simulink model "aerodynamic_model_V1_2_Wrench"  (R2025b)
settings: Solver=ode4  StartTime=0.0  StopTime=0.3  FixedStep=Ts  RelTol=1e-3
InitFcn:
  | % Run initial_main.m first to load Ad,As,Tq_prop,Tq_mass,...
values from neighbouring files (symbols this model uses):
  alpha_du0_v_tail_L = trim_aero_ic.v_tail_L.alpha_du0    [initial_main_V1_1.m]
  alpha_du0_v_tail_R = trim_aero_ic.v_tail_R.alpha_du0    [initial_main_V1_1.m]
  alpha_du0_wing_L = trim_aero_ic.wing_L.alpha_du0    [initial_main_V1_1.m]
  alpha_du0_wing_R = trim_aero_ic.wing_R.alpha_du0    [initial_main_V1_1.m]
  As = sys_sd.A    [initial_main_V1_1.m]
  BladePitch_deg = 34    [initial_main_V1_1.m]
  Bs = sys_sd.B    [initial_main_V1_1.m]
  Cs = sys_sd.C    [initial_main_V1_1.m]
  ctrl_delta_lim_deg = strips.delta_lim_deg    [initial_main_V1_1.m]
  ctrl_map_aileron_L = aero.wing_L.map_aileron(:)    [initial_main_V1_1.m]
  ctrl_map_aileron_R = aero.wing_R.map_aileron(:)    [initial_main_V1_1.m]
  ctrl_map_tail_L = aero.v_tail_L.map_tail(:)    [initial_main_V1_1.m]
  ctrl_map_tail_R = aero.v_tail_R.map_tail(:)    [initial_main_V1_1.m]
  Ds = sys_sd.D    [initial_main_V1_1.m]
  I_cg_b = R_sb * I_cg_m * R_sb.'    [aeroelastic.m]    (also in initial_main_V1_1.m = grav.I_cg_b)
  I_cg_b_inv = R_sb * I_cg_m_inv * R_sb.'    [aeroelastic.m]    (also in initial_main_V1_1.m = grav.I_cg_b_inv)
  m_node = zeros(n_id, 1)    [aeroelastic.m]    (also in generate_pullup_load_cloud.m = evalin('base', 'm_node(:)'); initial_main_V1_1.m = nodal.m_node)
  m_total_kg = evalin('base', 'm_total_kg')    [generate_pullup_load_cloud.m]    (also in initial_main_V1_1.m = grav.m_total_kg)
  n_modes = size(Phi, 2)    [aeroelastic.m]    (also in initial_main_V1_1.m = n_rigid + n_elastic)
  ones_1_tail = ones(1, size(r_cg2ac_b_v_tail_L, 2))    [initial_main_V1_1.m]
  ones_1_wing = ones(1, size(r_cg2ac_b_wing_L, 2))    [initial_main_V1_1.m]
  Phi = evalin('base', 'Phi')    [generate_pullup_load_cloud.m]    (also in initial_main_V1_1.m = strips.Phi)
  polar_alpha_deg = polar.alpha_deg(:).'    [initial_main_V1_1.m]
  polar_CD = polar.CD(:).'    [initial_main_V1_1.m]
  polar_CDp = polar.CDp(:).'    [initial_main_V1_1.m]
  polar_CL = polar.CL(:).'    [initial_main_V1_1.m]
  polar_CM = polar.CM(:).'    [initial_main_V1_1.m]
  r_cg2ac_b_v_tail_L = R_sb * aero.v_tail_L.r_ac_s    [initial_main_V1_1.m]
  r_cg2ac_b_v_tail_R = R_sb * aero.v_tail_R.r_ac_s    [initial_main_V1_1.m]
  r_cg2ac_b_wing_L = R_sb * aero.wing_L.r_ac_s    [initial_main_V1_1.m]
  r_cg2ac_b_wing_R = R_sb * aero.wing_R.r_ac_s    [initial_main_V1_1.m]
  r_cg2kink_b = eng.r_cg2kink_b    [initial_main_V1_1.m]
  r_cg2node_b = aeroelastic.node_arms(nodes, 'R_sb', R_sb).r_cg2node_b    [initial_main_V1_1.m]
  surface_nodes = aeroelastic.surface_load_nodes(nodes)    [initial_main_V1_1.m]
  T_aero2W = aeroelastic.wing_aileron_to_W(strips).T    [initial_main_V1_1.m]
  T_prop2W = load_maps.T_prop2W    [initial_main_V1_1.m]
  Tq_mass = load_maps.Tq_mass    [initial_main_V1_1.m]
  trim_Attitude_rad0 = trim_default.Attitude_rad0    [initial_main_V1_1.m]
  trim_Omega_b0 = trim_default.Omega_b0    [initial_main_V1_1.m]
  trim_Position0 = trim_default.Position0    [initial_main_V1_1.m]
  trim_Velocity_b0 = trim_default.Velocity_b0    [initial_main_V1_1.m]
  Ts = 0.001    [initial_main_V1_1.m]
  U = 55    [initial_main_V1_1.m]
  v_tail_cant_rad = deg2rad(v_tail_cant_deg)    [initial_main_V1_1.m]
  W_mass_g = grav.W_mass    [initial_main_V1_1.m]
  x0_structure = trim_default.x0_structure    [initial_main_V1_1.m]
  x0_wagner_v_tail_L = trim_aero_ic.v_tail_L.x0_wagner    [initial_main_V1_1.m]
  x0_wagner_v_tail_R = trim_aero_ic.v_tail_R.x0_wagner    [initial_main_V1_1.m]
  x0_wagner_wing_L = trim_aero_ic.wing_L.x0_wagner    [initial_main_V1_1.m]
  x0_wagner_wing_R = trim_aero_ic.wing_R.x0_wagner    [initial_main_V1_1.m]
undefined symbols (not defined in the file or in its folder): Ad_v_tail_L, Ad_v_tail_R, Ad_wing_L, Ad_wing_R, Bd_v_tail_L, Bd_v_tail_R, Bd_wing_L, Bd_wing_R, c_over_2U_v_tail_L, c_over_2U_v_tail_R, c_over_2U_wing_L, c_over_2U_wing_R, Cd_v_tail_L, Cd_v_tail_R, Cd_wing_L, Cd_wing_R, Dd_v_tail_L, Dd_v_tail_R, Dd_wing_L, Dd_wing_R, G_du_v_tail_L, G_du_v_tail_R, G_du_wing_L, G_du_wing_R, polar_aileron_alpha_deg, polar_aileron_dCD, polar_aileron_dCL, polar_aileron_dCM, polar_aileron_delta_deg, polar_ruddervator_alpha_deg, polar_ruddervator_dCD, polar_ruddervator_dCL, polar_ruddervator_dCM, polar_ruddervator_delta_deg, qS_strip_v_tail_L, qS_strip_v_tail_R, qS_strip_wing_L, qS_strip_wing_R, qSc_strip_v_tail_L, qSc_strip_v_tail_R, qSc_strip_wing_L, qSc_strip_wing_R, T_m2b_v_tail_L, T_m2b_v_tail_R, T_m2b_wing_L, T_m2b_wing_R, T_m2h_v_tail_L, T_m2h_v_tail_R, T_m2h_wing_L, T_m2h_wing_R, Tq_CM_v_tail_L, Tq_CM_v_tail_R, Tq_CM_wing_L, Tq_CM_wing_R, Tq_D_v_tail_L, Tq_D_v_tail_R, Tq_D_wing_L, Tq_D_wing_R, Tq_v_tail_L, Tq_v_tail_R ... (+2)
libraries: Prop_gryo x12, matrix_library x2
(part 4 of 6)

== system aerodynamic_model_V1_2_Wrench/Load Estimator/Engine_station/Subsystem7 ==
  In1 : Inport
  r_cg_up : Inport  Port=2
  Bus Creator : BusCreator  Inputs=6
  Bus Creator1 : BusCreator  Inputs=6
  Bus Creator2 : BusCreator  Inputs=6
  Bus Creator4 : BusCreator  Inputs=3
  Constant : Constant  Value=r_cg2node_b(:,67)
  Constant1 : Constant  Value=r_cg2node_b(:,66)
  Constant2 : Constant  Value=0
  Constant3 : Constant  Value=r_cg2node_b(:,46)
  Constant4 : Constant  Value=[0 0 0]/180*pi
  Constant5 : Constant  Value=[-7 0 0]/180*pi
  Constant6 : Constant  Value=-7
  Constant7 : Constant  Value=90
  Demux{1..6} (6 alike) : Demux  Outputs=3
  Gain : Gain  Gain=pi/180
  MATLAB Function1 : MATLAB Function  TreatAsAtomicUnit=on
  MATLAB Function2 : MATLAB Function  TreatAsAtomicUnit=on
  MATLAB Function3 : MATLAB Function  TreatAsAtomicUnit=on
  Mux : Mux  Inputs=3
  Product{1..4,6..7} (6 alike) : Product  Multiplication=Matrix(*)
  Rotation Angles to Direction Cosine Matrix : Angle2Dcm  rotationOrder=XYZ
      settings: AttributesFormatString=Rotation Order: %<rotationOrder>
  Rotation Angles to Direction Cosine Matrix1 : Angle2Dcm  rotationOrder=XYZ
      settings: AttributesFormatString=Rotation Order: %<rotationOrder>
  Rotation Angles to Direction Cosine Matrix2 : Angle2Dcm  rotationOrder=XYZ
      settings: AttributesFormatString=Rotation Order: %<rotationOrder>
  Selector1 : Selector  NumberOfDimensions=2  InputPortWidth=3  IndexOptions=Select all,Index vector (dialog)  Indices=[1:6],[67]  OutputSizes=1,1
  Selector10 : Selector  NumberOfDimensions=2  InputPortWidth=3  IndexOptions=Index vector (dialog),Select all  Indices=[4:6],[surface_nodes.wing_R.node_id]  OutputSizes=1,1
  Selector11 : Selector  NumberOfDimensions=2  InputPortWidth=3  IndexOptions=Index vector (dialog),Select all  Indices=[4:6],[surface_nodes.wing_R.node_id]  OutputSizes=1,1
  Selector12 : Selector  NumberOfDimensions=2  InputPortWidth=3  IndexOptions=Index vector (dialog),Select all  Indices=[1:3],[surface_nodes.wing_R.node_id]  OutputSizes=1,1
  Selector13 : Selector  NumberOfDimensions=2  InputPortWidth=3  IndexOptions=Index vector (dialog),Select all  Indices=[4:6],[surface_nodes.wing_R.node_id]  OutputSizes=1,1
  Selector14 : Selector  NumberOfDimensions=2  InputPortWidth=3  IndexOptions=Index vector (dialog),Select all  Indices=[1:3],[surface_nodes.wing_R.node_id]  OutputSizes=1,1
  Selector2 : Selector  NumberOfDimensions=2  InputPortWidth=3  IndexOptions=Select all,Index vector (dialog)  Indices=[1:6],[66 67]  OutputSizes=1,1
  Selector3 : Selector  NumberOfDimensions=2  InputPortWidth=3  IndexOptions=Select all,Index vector (dialog)  Indices=[1:6],[67]  OutputSizes=1,1
  Selector4 : Selector  NumberOfDimensions=2  InputPortWidth=3  IndexOptions=Select all,Index vector (dialog)  Indices=[1:6],[66 67]  OutputSizes=1,1
  Selector5 : Selector  NumberOfDimensions=2  InputPortWidth=3  IndexOptions=Select all,Index vector (dialog)  Indices=[1:6],[65:67]  OutputSizes=1,1
  Selector6 : Selector  NumberOfDimensions=2  InputPortWidth=3  IndexOptions=Select all,Index vector (dialog)  Indices=[1:6],[65:67]  OutputSizes=1,1
  Selector9 : Selector  NumberOfDimensions=2  InputPortWidth=3  IndexOptions=Index vector (dialog),Select all  Indices=[1:3],[surface_nodes.wing_R.node_id]  OutputSizes=1,1
  Out1 : Outport
  wires:
  Demux3/3 -> Bus Creator2/3  "shear_forcez"
  Selector4/1 -> MATLAB Function2/3(r)
  MATLAB Function3/2(M_b) -> Product4/2
  MATLAB Function1/2(M_b) -> Product7/2
  Demux1/2 -> Bus Creator1/2  "shear_forcey"
  Demux6/3 -> Bus Creator2/6  "Bending_momenty"
  MATLAB Function1/1(F_b) -> Product6/2
  Selector6/1 -> MATLAB Function3/3(r)
  Demux1/3 -> Bus Creator1/3  "shear_forcez"
  Demux5/2 -> Bus Creator/5  "Bending_momentx"
  Selector2/1 -> Selector11/1, Selector12/1
  Demux4/2 -> Bus Creator/2  "shear_forcey"
  Selector12/1 -> MATLAB Function2/1(F)
  Bus Creator1/1 -> Bus Creator4/2
  Demux5/3 -> Bus Creator/6  "Bending_momenty"
  Selector5/1 -> Selector13/1, Selector14/1
  Constant1/1 -> MATLAB Function2/4(p)
  Demux5/1 -> Bus Creator/4  "Torision_moment"
  Constant2/1 -> Mux/3
  Gain/1 -> Rotation Angles to Direction Cosine Matrix/1
  Bus Creator2/1 -> Bus Creator4/3
  Product3/1 -> Demux3/1
  Demux1/1 -> Bus Creator1/1  "Axial_Force"
  Selector9/1 -> MATLAB Function1/1(F)
  Product7/1 -> Demux5/1
  Bus Creator/1 -> Bus Creator4/1
  Demux4/1 -> Bus Creator/1  "Axial_Force"
  In1/1 -> Selector1/1, Selector5/1, Selector2/1
  Demux2/1 -> Bus Creator1/4  "Torision_moment"
  Rotation Angles to Direction Cosine Matrix2/1 -> Product4/1, Product3/1
  Constant6/1 -> Mux/1
  Mux/1 -> Gain/1
  Product6/1 -> Demux4/1
  Demux3/1 -> Bus Creator2/1  "Axial_Force"
  Selector11/1 -> MATLAB Function2/2(M)
  Demux6/1 -> Bus Creator2/4  "Torision_moment"
  Demux2/3 -> Bus Creator1/6  "Bending_momenty"
  MATLAB Function2/1(F_b) -> Product1/2
  Rotation Angles to Direction Cosine Matrix1/1 -> Product1/1, Product2/1
  Demux4/3 -> Bus Creator/3  "shear_forcez"
  Constant3/1 -> MATLAB Function3/4(p)
  Product1/1 -> Demux1/1
  Product2/1 -> Demux2/1
  Constant5/1 -> Rotation Angles to Direction Cosine Matrix1/1
  MATLAB Function2/2(M_b) -> Product2/2
  Bus Creator4/1 -> Out1/1
  r_cg_up/1 -> Selector6/1, Selector4/1, Selector3/1
  Selector1/1 -> Selector10/1, Selector9/1
  MATLAB Function3/1(F_b) -> Product3/2
  Constant7/1 -> Mux/2
  Selector10/1 -> MATLAB Function1/2(M)
  Rotation Angles to Direction Cosine Matrix/1 -> Product7/1, Product6/1
  Selector13/1 -> MATLAB Function3/2(M)
  Constant4/1 -> Rotation Angles to Direction Cosine Matrix2/1
  Selector14/1 -> MATLAB Function3/1(F)
  Demux2/2 -> Bus Creator1/5  "Bending_momentx"
  Demux3/2 -> Bus Creator2/2  "shear_forcey"
  Selector3/1 -> MATLAB Function1/3(r)
  Constant/1 -> MATLAB Function1/4(p)
  Demux6/2 -> Bus Creator2/5  "Bending_momentx"
  Product4/1 -> Demux6/1

== system aerodynamic_model_V1_2_Wrench/Load Estimator/Engine_station1/Subsystem ==
  In1 : Inport
  In2 : Inport  Port=2
  Bus Creator : BusCreator  Inputs=6
  Bus Creator1 : BusCreator  Inputs=6
  Bus Creator2 : BusCreator  Inputs=6
  Bus Creator4 : BusCreator  Inputs=3
  Constant : Constant  Value=r_cg2node_b(:,76)
  Constant1 : Constant  Value=r_cg2node_b(:,75)
  Constant2 : Constant  Value=0
  Constant3 : Constant  Value=r_cg2node_b(:,47)
  Constant4 : Constant  Value=[0 0 0]/180*pi
  Constant5 : Constant  Value=[-7 0 0]/180*pi
  Constant6 : Constant  Value=-7
  Constant7 : Constant  Value=90
  Demux{1..6} (6 alike) : Demux  Outputs=3
  Gain : Gain  Gain=pi/180
  MATLAB Function1 : MATLAB Function  TreatAsAtomicUnit=on
  MATLAB Function2 : MATLAB Function  TreatAsAtomicUnit=on
  MATLAB Function3 : MATLAB Function  TreatAsAtomicUnit=on
  Mux : Mux  Inputs=3
  Product{1..4,6..7} (6 alike) : Product  Multiplication=Matrix(*)
  Rotation Angles to Direction Cosine Matrix : Angle2Dcm  rotationOrder=XYZ
      settings: AttributesFormatString=Rotation Order: %<rotationOrder>
  Rotation Angles to Direction Cosine Matrix1 : Angle2Dcm  rotationOrder=XYZ
      settings: AttributesFormatString=Rotation Order: %<rotationOrder>
  Rotation Angles to Direction Cosine Matrix2 : Angle2Dcm  rotationOrder=XYZ
      settings: AttributesFormatString=Rotation Order: %<rotationOrder>
  Selector1 : Selector  NumberOfDimensions=2  InputPortWidth=3  IndexOptions=Select all,Index vector (dialog)  Indices=[1:6],[75 76]  OutputSizes=1,1
  Selector10 : Selector  NumberOfDimensions=2  InputPortWidth=3  IndexOptions=Index vector (dialog),Select all  Indices=[4:6],[surface_nodes.wing_R.node_id]  OutputSizes=1,1
  Selector11 : Selector  NumberOfDimensions=2  InputPortWidth=3  IndexOptions=Index vector (dialog),Select all  Indices=[4:6],[surface_nodes.wing_R.node_id]  OutputSizes=1,1
  Selector12 : Selector  NumberOfDimensions=2  InputPortWidth=3  IndexOptions=Index vector (dialog),Select all  Indices=[1:3],[surface_nodes.wing_R.node_id]  OutputSizes=1,1
  Selector13 : Selector  NumberOfDimensions=2  InputPortWidth=3  IndexOptions=Index vector (dialog),Select all  Indices=[4:6],[surface_nodes.wing_R.node_id]  OutputSizes=1,1
  Selector14 : Selector  NumberOfDimensions=2  InputPortWidth=3  IndexOptions=Index vector (dialog),Select all  Indices=[1:3],[surface_nodes.wing_R.node_id]  OutputSizes=1,1
  Selector2 : Selector  NumberOfDimensions=2  InputPortWidth=3  IndexOptions=Select all,Index vector (dialog)  Indices=[1:6],[76]  OutputSizes=1,1
  Selector3 : Selector  NumberOfDimensions=2  InputPortWidth=3  IndexOptions=Select all,Index vector (dialog)  Indices=[1:6],[76]  OutputSizes=1,1
  Selector4 : Selector  NumberOfDimensions=2  InputPortWidth=3  IndexOptions=Select all,Index vector (dialog)  Indices=[1:6],[75 76]  OutputSizes=1,1
  Selector5 : Selector  NumberOfDimensions=2  InputPortWidth=3  IndexOptions=Select all,Index vector (dialog)  Indices=[1:6],[74:76]  OutputSizes=1,1
  Selector6 : Selector  NumberOfDimensions=2  InputPortWidth=3  IndexOptions=Select all,Index vector (dialog)  Indices=[1:6],[74:76]  OutputSizes=1,1
  Selector9 : Selector  NumberOfDimensions=2  InputPortWidth=3  IndexOptions=Index vector (dialog),Select all  Indices=[1:3],[surface_nodes.wing_R.node_id]  OutputSizes=1,1
  Out1 : Outport
  wires:
  Demux3/3 -> Bus Creator2/3  "shear_forcez"
  Selector4/1 -> MATLAB Function2/3(r)
  MATLAB Function3/2(M_b) -> Product4/2
  MATLAB Function1/2(M_b) -> Product7/2
  Demux1/2 -> Bus Creator1/2  "shear_forcey"
  Demux6/3 -> Bus Creator2/6  "Bending_momenty"
  MATLAB Function1/1(F_b) -> Product6/2
  Selector6/1 -> MATLAB Function3/3(r)
  Demux1/3 -> Bus Creator1/3  "shear_forcez"
  Demux5/2 -> Bus Creator/5  "Bending_momentx"
  Selector1/1 -> Selector11/1, Selector12/1
  Demux4/2 -> Bus Creator/2  "shear_forcey"
  Selector12/1 -> MATLAB Function2/1(F)
  Bus Creator1/1 -> Bus Creator4/2
  Demux5/3 -> Bus Creator/6  "Bending_momenty"
  Selector5/1 -> Selector13/1, Selector14/1
  Constant1/1 -> MATLAB Function2/4(p)
  Demux5/1 -> Bus Creator/4  "Torision_moment"
  Constant2/1 -> Mux/3
  Gain/1 -> Rotation Angles to Direction Cosine Matrix/1
  Bus Creator2/1 -> Bus Creator4/3
  Product3/1 -> Demux3/1
  Demux1/1 -> Bus Creator1/1  "Axial_Force"
  Selector9/1 -> MATLAB Function1/1(F)
  Product7/1 -> Demux5/1
  Bus Creator/1 -> Bus Creator4/1
  Demux4/1 -> Bus Creator/1  "Axial_Force"
  In1/1 -> Selector1/1, Selector5/1, Selector2/1
  Demux2/1 -> Bus Creator1/4  "Torision_moment"
  Rotation Angles to Direction Cosine Matrix2/1 -> Product4/1, Product3/1
  Constant6/1 -> Mux/1
  Mux/1 -> Gain/1
  Product6/1 -> Demux4/1
  Demux3/1 -> Bus Creator2/1  "Axial_Force"
  Selector11/1 -> MATLAB Function2/2(M)
  Demux6/1 -> Bus Creator2/4  "Torision_moment"
  Demux2/3 -> Bus Creator1/6  "Bending_momenty"
  MATLAB Function2/1(F_b) -> Product1/2
  Rotation Angles to Direction Cosine Matrix1/1 -> Product1/1, Product2/1
  Demux4/3 -> Bus Creator/3  "shear_forcez"
  Constant3/1 -> MATLAB Function3/4(p)
  Product1/1 -> Demux1/1
  Product2/1 -> Demux2/1
  Constant5/1 -> Rotation Angles to Direction Cosine Matrix1/1
  MATLAB Function2/2(M_b) -> Product2/2
  Bus Creator4/1 -> Out1/1
  In2/1 -> Selector6/1, Selector4/1, Selector3/1
  Selector2/1 -> Selector10/1, Selector9/1
  MATLAB Function3/1(F_b) -> Product3/2
  Constant7/1 -> Mux/2
  Selector10/1 -> MATLAB Function1/2(M)
  Rotation Angles to Direction Cosine Matrix/1 -> Product7/1, Product6/1
  Selector13/1 -> MATLAB Function3/2(M)
  Constant4/1 -> Rotation Angles to Direction Cosine Matrix2/1
  Selector14/1 -> MATLAB Function3/1(F)
  Demux2/2 -> Bus Creator1/5  "Bending_momentx"
  Demux3/2 -> Bus Creator2/2  "shear_forcey"
  Selector3/1 -> MATLAB Function1/3(r)
  Constant/1 -> MATLAB Function1/4(p)
  Demux6/2 -> Bus Creator2/5  "Bending_momentx"
  Product4/1 -> Demux6/1

== system aerodynamic_model_V1_2_Wrench/Load Estimator/Engine_station1/Subsystem1 ==
  Wb_total : Inport
  r_cg_up : Inport  Port=2
  tilt_deg : Inport  Port=3
  Bus Creator : BusCreator  Inputs=6
  Bus Creator1 : BusCreator  Inputs=6
  Bus Creator2 : BusCreator  Inputs=6
  Bus Creator4 : BusCreator  Inputs=3
  Constant : Constant  Value=r_cg2node_b(:,70)
  Constant1 : Constant  Value=r_cg2node_b(:,69)
  Constant2 : Constant  Value=0
  Constant3 : Constant  Value=r_cg2node_b(:,29)
  Constant4 : Constant  Value=[0 0 0]/180*pi
  Constant5 : Constant  Value=[-7 0 0]/180*pi
  Constant6 : Constant  Value=-7
  Demux{1..6} (6 alike) : Demux  Outputs=3
  Gain : Gain  Gain=pi/180
  MATLAB Function1 : MATLAB Function  TreatAsAtomicUnit=on
  MATLAB Function2 : MATLAB Function  TreatAsAtomicUnit=on
  MATLAB Function3 : MATLAB Function  TreatAsAtomicUnit=on
  Mux : Mux  Inputs=3
  Product{1..4,6..7} (6 alike) : Product  Multiplication=Matrix(*)
  Rotation Angles to Direction Cosine Matrix : Angle2Dcm
      settings: AttributesFormatString=Rotation Order: %<rotationOrder>
  Rotation Angles to Direction Cosine Matrix1 : Angle2Dcm
      settings: AttributesFormatString=Rotation Order: %<rotationOrder>
  Rotation Angles to Direction Cosine Matrix2 : Angle2Dcm
      settings: AttributesFormatString=Rotation Order: %<rotationOrder>
  Selector1 : Selector  NumberOfDimensions=2  InputPortWidth=3  IndexOptions=Select all,Index vector (dialog)  Indices=[1:6],[69 70]  OutputSizes=1,1
  Selector10 : Selector  NumberOfDimensions=2  InputPortWidth=3  IndexOptions=Index vector (dialog),Select all  Indices=[4:6],[surface_nodes.wing_R.node_id]  OutputSizes=1,1
  Selector11 : Selector  NumberOfDimensions=2  InputPortWidth=3  IndexOptions=Index vector (dialog),Select all  Indices=[4:6],[surface_nodes.wing_R.node_id]  OutputSizes=1,1
  Selector12 : Selector  NumberOfDimensions=2  InputPortWidth=3  IndexOptions=Index vector (dialog),Select all  Indices=[1:3],[surface_nodes.wing_R.node_id]  OutputSizes=1,1
  Selector13 : Selector  NumberOfDimensions=2  InputPortWidth=3  IndexOptions=Index vector (dialog),Select all  Indices=[4:6],[surface_nodes.wing_R.node_id]  OutputSizes=1,1
  Selector14 : Selector  NumberOfDimensions=2  InputPortWidth=3  IndexOptions=Index vector (dialog),Select all  Indices=[1:3],[surface_nodes.wing_R.node_id]  OutputSizes=1,1
  Selector2 : Selector  NumberOfDimensions=2  InputPortWidth=3  IndexOptions=Select all,Index vector (dialog)  Indices=[1:6],[70]  OutputSizes=1,1
  Selector3 : Selector  NumberOfDimensions=2  InputPortWidth=3  IndexOptions=Select all,Index vector (dialog)  Indices=[1:6],[70]  OutputSizes=1,1
  Selector4 : Selector  NumberOfDimensions=2  InputPortWidth=3  IndexOptions=Select all,Index vector (dialog)  Indices=[1:6],[69 70]  OutputSizes=1,1
  Selector5 : Selector  NumberOfDimensions=2  InputPortWidth=3  IndexOptions=Select all,Index vector (dialog)  Indices=[1:6],[68:70]  OutputSizes=1,1
  Selector6 : Selector  NumberOfDimensions=2  InputPortWidth=3  IndexOptions=Select all,Index vector (dialog)  Indices=[1:6],[68:70]  OutputSizes=1,1
  Selector9 : Selector  NumberOfDimensions=2  InputPortWidth=3  IndexOptions=Index vector (dialog),Select all  Indices=[1:3],[surface_nodes.wing_R.node_id]  OutputSizes=1,1
  Out1 : Outport
  wires:
  Product4/1 -> Demux6/1
  Demux6/2 -> Bus Creator2/5  "Bending_momentx"
  Constant/1 -> MATLAB Function1/4(p)
  Selector3/1 -> MATLAB Function1/3(r)
  Demux3/2 -> Bus Creator2/2  "shear_forcey"
  Demux2/2 -> Bus Creator1/5  "Bending_momentx"
  Selector14/1 -> MATLAB Function3/1(F)
  Constant4/1 -> Rotation Angles to Direction Cosine Matrix2/1
  Selector13/1 -> MATLAB Function3/2(M)
  Rotation Angles to Direction Cosine Matrix/1 -> Product6/1, Product7/1
  Selector10/1 -> MATLAB Function1/2(M)
  tilt_deg/1 -> Mux/2
  MATLAB Function3/1(F_b) -> Product3/2
  Selector2/1 -> Selector9/1, Selector10/1
  r_cg_up/1 -> Selector3/1, Selector4/1, Selector6/1
  Bus Creator4/1 -> Out1/1
  MATLAB Function2/2(M_b) -> Product2/2
  Constant5/1 -> Rotation Angles to Direction Cosine Matrix1/1
  Product2/1 -> Demux2/1
  Product1/1 -> Demux1/1
  Constant3/1 -> MATLAB Function3/4(p)
  Demux4/3 -> Bus Creator/3  "shear_forcez"
  Rotation Angles to Direction Cosine Matrix1/1 -> Product2/1, Product1/1
  MATLAB Function2/1(F_b) -> Product1/2
  Demux2/3 -> Bus Creator1/6  "Bending_momenty"
  Demux6/1 -> Bus Creator2/4  "Torision_moment"
  Selector11/1 -> MATLAB Function2/2(M)
  Demux3/1 -> Bus Creator2/1  "Axial_Force"
  Product6/1 -> Demux4/1
  Mux/1 -> Gain/1
  Constant6/1 -> Mux/1
  Rotation Angles to Direction Cosine Matrix2/1 -> Product3/1, Product4/1
  Demux2/1 -> Bus Creator1/4  "Torision_moment"
  Wb_total/1 -> Selector5/1, Selector1/1, Selector2/1
  Demux4/1 -> Bus Creator/1  "Axial_Force"
  Bus Creator/1 -> Bus Creator4/1
  Product7/1 -> Demux5/1
  Selector9/1 -> MATLAB Function1/1(F)
  Demux1/1 -> Bus Creator1/1  "Axial_Force"
  Product3/1 -> Demux3/1
  Bus Creator2/1 -> Bus Creator4/3
  Gain/1 -> Rotation Angles to Direction Cosine Matrix/1
  Constant2/1 -> Mux/3
  Demux5/1 -> Bus Creator/4  "Torision_moment"
  Constant1/1 -> MATLAB Function2/4(p)
  Selector5/1 -> Selector14/1, Selector13/1
  Demux5/3 -> Bus Creator/6  "Bending_momenty"
  Bus Creator1/1 -> Bus Creator4/2
  Selector12/1 -> MATLAB Function2/1(F)
  Demux4/2 -> Bus Creator/2  "shear_forcey"
  Selector1/1 -> Selector12/1, Selector11/1
  Demux5/2 -> Bus Creator/5  "Bending_momentx"
  Demux1/3 -> Bus Creator1/3  "shear_forcez"
  Selector6/1 -> MATLAB Function3/3(r)
  MATLAB Function1/1(F_b) -> Product6/2
  Demux6/3 -> Bus Creator2/6  "Bending_momenty"
  Demux1/2 -> Bus Creator1/2  "shear_forcey"
  MATLAB Function1/2(M_b) -> Product7/2
  MATLAB Function3/2(M_b) -> Product4/2
  Selector4/1 -> MATLAB Function2/3(r)
  Demux3/3 -> Bus Creator2/3  "shear_forcez"

== system aerodynamic_model_V1_2_Wrench/Load Estimator/Engine_station1/Subsystem2 ==
  Wb_total : Inport
  r_cg_up : Inport  Port=2
  In3 : Inport  Port=3
  Bus Creator : BusCreator  Inputs=6
  Bus Creator1 : BusCreator  Inputs=6
  Bus Creator2 : BusCreator  Inputs=6
  Bus Creator4 : BusCreator  Inputs=3
  Constant : Constant  Value=r_cg2node_b(:,58)
  Constant1 : Constant  Value=r_cg2node_b(:,57)
  Constant2 : Constant  Value=0
  Constant3 : Constant  Value=r_cg2node_b(:,28)
  Constant4 : Constant  Value=[0 0 0]/180*pi
  Constant5 : Constant  Value=[7 0 0]/180*pi
  Constant6 : Constant  Value=7
  Demux{1..6} (6 alike) : Demux  Outputs=3
  Gain : Gain  Gain=pi/180
  MATLAB Function1 : MATLAB Function  TreatAsAtomicUnit=on
  MATLAB Function2 : MATLAB Function  TreatAsAtomicUnit=on
  MATLAB Function3 : MATLAB Function  TreatAsAtomicUnit=on
  Mux : Mux  Inputs=3
  Product{1..4,6..7} (6 alike) : Product  Multiplication=Matrix(*)
  Rotation Angles to Direction Cosine Matrix : Angle2Dcm  rotationOrder=XYZ
      settings: AttributesFormatString=Rotation Order: %<rotationOrder>
  Rotation Angles to Direction Cosine Matrix1 : Angle2Dcm  rotationOrder=XYZ
      settings: AttributesFormatString=Rotation Order: %<rotationOrder>
  Rotation Angles to Direction Cosine Matrix2 : Angle2Dcm  rotationOrder=XYZ
      settings: AttributesFormatString=Rotation Order: %<rotationOrder>
  Selector1 : Selector  NumberOfDimensions=2  InputPortWidth=3  IndexOptions=Select all,Index vector (dialog)  Indices=[1:6],[57 58]  OutputSizes=1,1
  Selector10 : Selector  NumberOfDimensions=2  InputPortWidth=3  IndexOptions=Index vector (dialog),Select all  Indices=[4:6],[surface_nodes.wing_R.node_id]  OutputSizes=1,1
  Selector11 : Selector  NumberOfDimensions=2  InputPortWidth=3  IndexOptions=Index vector (dialog),Select all  Indices=[4:6],[surface_nodes.wing_R.node_id]  OutputSizes=1,1
  Selector12 : Selector  NumberOfDimensions=2  InputPortWidth=3  IndexOptions=Index vector (dialog),Select all  Indices=[1:3],[surface_nodes.wing_R.node_id]  OutputSizes=1,1
  Selector13 : Selector  NumberOfDimensions=2  InputPortWidth=3  IndexOptions=Index vector (dialog),Select all  Indices=[4:6],[surface_nodes.wing_R.node_id]  OutputSizes=1,1
  Selector14 : Selector  NumberOfDimensions=2  InputPortWidth=3  IndexOptions=Index vector (dialog),Select all  Indices=[1:3],[surface_nodes.wing_R.node_id]  OutputSizes=1,1
  Selector2 : Selector  NumberOfDimensions=2  InputPortWidth=3  IndexOptions=Select all,Index vector (dialog)  Indices=[1:6],[58]  OutputSizes=1,1
  Selector3 : Selector  NumberOfDimensions=2  InputPortWidth=3  IndexOptions=Select all,Index vector (dialog)  Indices=[1:6],[58]  OutputSizes=1,1
  Selector4 : Selector  NumberOfDimensions=2  InputPortWidth=3  IndexOptions=Select all,Index vector (dialog)  Indices=[1:6],[57 58]  OutputSizes=1,1
  Selector5 : Selector  NumberOfDimensions=2  InputPortWidth=3  IndexOptions=Select all,Index vector (dialog)  Indices=[1:6],[56:58]  OutputSizes=1,1
  Selector6 : Selector  NumberOfDimensions=2  InputPortWidth=3  IndexOptions=Select all,Index vector (dialog)  Indices=[1:6],[56:58]  OutputSizes=1,1
  Selector9 : Selector  NumberOfDimensions=2  InputPortWidth=3  IndexOptions=Index vector (dialog),Select all  Indices=[1:3],[surface_nodes.wing_R.node_id]  OutputSizes=1,1
  Out1 : Outport
  wires:
  Demux3/3 -> Bus Creator2/3  "shear_forcez"
  Selector4/1 -> MATLAB Function2/3(r)
  MATLAB Function3/2(M_b) -> Product4/2
  MATLAB Function1/2(M_b) -> Product7/2
  Demux1/2 -> Bus Creator1/2  "shear_forcey"
  Demux6/3 -> Bus Creator2/6  "Bending_momenty"
  MATLAB Function1/1(F_b) -> Product6/2
  Selector6/1 -> MATLAB Function3/3(r)
  Demux1/3 -> Bus Creator1/3  "shear_forcez"
  Demux5/2 -> Bus Creator/5  "Bending_momentx"
  Selector1/1 -> Selector11/1, Selector12/1
  Demux4/2 -> Bus Creator/2  "shear_forcey"
  Selector12/1 -> MATLAB Function2/1(F)
  Bus Creator1/1 -> Bus Creator4/2
  Demux5/3 -> Bus Creator/6  "Bending_momenty"
  Selector5/1 -> Selector13/1, Selector14/1
  Constant1/1 -> MATLAB Function2/4(p)
  Demux5/1 -> Bus Creator/4  "Torision_moment"
  Constant2/1 -> Mux/3
  Gain/1 -> Rotation Angles to Direction Cosine Matrix/1
  Bus Creator2/1 -> Bus Creator4/3
  Product3/1 -> Demux3/1
  Demux1/1 -> Bus Creator1/1  "Axial_Force"
  Selector9/1 -> MATLAB Function1/1(F)
  Product7/1 -> Demux5/1
  Bus Creator/1 -> Bus Creator4/1
  Demux4/1 -> Bus Creator/1  "Axial_Force"
  Wb_total/1 -> Selector5/1, Selector1/1, Selector2/1
  Demux2/1 -> Bus Creator1/4  "Torision_moment"
  Rotation Angles to Direction Cosine Matrix2/1 -> Product4/1, Product3/1
  Constant6/1 -> Mux/1
  Mux/1 -> Gain/1
  Product6/1 -> Demux4/1
  Demux3/1 -> Bus Creator2/1  "Axial_Force"
  Selector11/1 -> MATLAB Function2/2(M)
  Demux6/1 -> Bus Creator2/4  "Torision_moment"
  Demux2/3 -> Bus Creator1/6  "Bending_momenty"
  MATLAB Function2/1(F_b) -> Product1/2
  Rotation Angles to Direction Cosine Matrix1/1 -> Product1/1, Product2/1
  Demux4/3 -> Bus Creator/3  "shear_forcez"
  Constant3/1 -> MATLAB Function3/4(p)
  Product1/1 -> Demux1/1
  Product2/1 -> Demux2/1
  Constant5/1 -> Rotation Angles to Direction Cosine Matrix1/1
  MATLAB Function2/2(M_b) -> Product2/2
  Bus Creator4/1 -> Out1/1
  r_cg_up/1 -> Selector6/1, Selector4/1, Selector3/1
  Selector2/1 -> Selector10/1, Selector9/1
  MATLAB Function3/1(F_b) -> Product3/2
  In3/1 -> Mux/2
  Selector10/1 -> MATLAB Function1/2(M)
  Rotation Angles to Direction Cosine Matrix/1 -> Product7/1, Product6/1
  Selector13/1 -> MATLAB Function3/2(M)
  Constant4/1 -> Rotation Angles to Direction Cosine Matrix2/1
  Selector14/1 -> MATLAB Function3/1(F)
  Demux2/2 -> Bus Creator1/5  "Bending_momentx"
  Demux3/2 -> Bus Creator2/2  "shear_forcey"
  Selector3/1 -> MATLAB Function1/3(r)
  Constant/1 -> MATLAB Function1/4(p)
  Demux6/2 -> Bus Creator2/5  "Bending_momentx"
  Product4/1 -> Demux6/1

== system aerodynamic_model_V1_2_Wrench/Load Estimator/Engine_station1/Subsystem3 ==
  In1 : Inport
  r_cg_up : Inport  Port=2
  Bus Creator : BusCreator  Inputs=6
  Bus Creator1 : BusCreator  Inputs=6
  Bus Creator2 : BusCreator  Inputs=6
  Bus Creator4 : BusCreator  Inputs=3
  Constant : Constant  Value=r_cg2node_b(:,64)
  Constant1 : Constant  Value=r_cg2node_b(:,63)
  Constant2 : Constant  Value=0
  Constant3 : Constant  Value=r_cg2node_b(:,46)
  Constant4 : Constant  Value=[0 0 0]/180*pi
  Constant5 : Constant  Value=[7 0 0]/180*pi
  Constant6 : Constant  Value=7
  Constant7 : Constant  Value=90
  Demux{1..6} (6 alike) : Demux  Outputs=3
  Gain : Gain  Gain=pi/180
  MATLAB Function1 : MATLAB Function  TreatAsAtomicUnit=on
  MATLAB Function2 : MATLAB Function  TreatAsAtomicUnit=on
  MATLAB Function3 : MATLAB Function  TreatAsAtomicUnit=on
  Mux : Mux  Inputs=3
  Product{1..4,6..7} (6 alike) : Product  Multiplication=Matrix(*)
  Rotation Angles to Direction Cosine Matrix : Angle2Dcm  rotationOrder=XYZ
      settings: AttributesFormatString=Rotation Order: %<rotationOrder>
  Rotation Angles to Direction Cosine Matrix1 : Angle2Dcm  rotationOrder=XYZ
      settings: AttributesFormatString=Rotation Order: %<rotationOrder>
  Rotation Angles to Direction Cosine Matrix2 : Angle2Dcm  rotationOrder=XYZ
      settings: AttributesFormatString=Rotation Order: %<rotationOrder>
  Selector1 : Selector  NumberOfDimensions=2  InputPortWidth=3  IndexOptions=Select all,Index vector (dialog)  Indices=[1:6],[63 64]  OutputSizes=1,1
  Selector10 : Selector  NumberOfDimensions=2  InputPortWidth=3  IndexOptions=Index vector (dialog),Select all  Indices=[4:6],[surface_nodes.wing_R.node_id]  OutputSizes=1,1
  Selector11 : Selector  NumberOfDimensions=2  InputPortWidth=3  IndexOptions=Index vector (dialog),Select all  Indices=[4:6],[surface_nodes.wing_R.node_id]  OutputSizes=1,1
  Selector12 : Selector  NumberOfDimensions=2  InputPortWidth=3  IndexOptions=Index vector (dialog),Select all  Indices=[1:3],[surface_nodes.wing_R.node_id]  OutputSizes=1,1
  Selector13 : Selector  NumberOfDimensions=2  InputPortWidth=3  IndexOptions=Index vector (dialog),Select all  Indices=[4:6],[surface_nodes.wing_R.node_id]  OutputSizes=1,1
  Selector14 : Selector  NumberOfDimensions=2  InputPortWidth=3  IndexOptions=Index vector (dialog),Select all  Indices=[1:3],[surface_nodes.wing_R.node_id]  OutputSizes=1,1
  Selector2 : Selector  NumberOfDimensions=2  InputPortWidth=3  IndexOptions=Select all,Index vector (dialog)  Indices=[1:6],[64]  OutputSizes=1,1
  Selector3 : Selector  NumberOfDimensions=2  InputPortWidth=3  IndexOptions=Select all,Index vector (dialog)  Indices=[1:6],[64]  OutputSizes=1,1
  Selector4 : Selector  NumberOfDimensions=2  InputPortWidth=3  IndexOptions=Select all,Index vector (dialog)  Indices=[1:6],[63 64]  OutputSizes=1,1
  Selector5 : Selector  NumberOfDimensions=2  InputPortWidth=3  IndexOptions=Select all,Index vector (dialog)  Indices=[1:6],[62:64]  OutputSizes=1,1
  Selector6 : Selector  NumberOfDimensions=2  InputPortWidth=3  IndexOptions=Select all,Index vector (dialog)  Indices=[1:6],[62:64]  OutputSizes=1,1
  Selector9 : Selector  NumberOfDimensions=2  InputPortWidth=3  IndexOptions=Index vector (dialog),Select all  Indices=[1:3],[surface_nodes.wing_R.node_id]  OutputSizes=1,1
  Out1 : Outport
  wires:
  Product4/1 -> Demux6/1
  Demux6/2 -> Bus Creator2/5  "Bending_momentx"
  Constant/1 -> MATLAB Function1/4(p)
  Selector3/1 -> MATLAB Function1/3(r)
  Demux3/2 -> Bus Creator2/2  "shear_forcey"
  Demux2/2 -> Bus Creator1/5  "Bending_momentx"
  Selector14/1 -> MATLAB Function3/1(F)
  Constant4/1 -> Rotation Angles to Direction Cosine Matrix2/1
  Selector13/1 -> MATLAB Function3/2(M)
  Rotation Angles to Direction Cosine Matrix/1 -> Product6/1, Product7/1
  Selector10/1 -> MATLAB Function1/2(M)
  Constant7/1 -> Mux/2
  MATLAB Function3/1(F_b) -> Product3/2
  Selector2/1 -> Selector9/1, Selector10/1
  r_cg_up/1 -> Selector6/1, Selector4/1, Selector3/1
  Bus Creator4/1 -> Out1/1
  MATLAB Function2/2(M_b) -> Product2/2
  Constant5/1 -> Rotation Angles to Direction Cosine Matrix1/1
  Product2/1 -> Demux2/1
  Product1/1 -> Demux1/1
  Constant3/1 -> MATLAB Function3/4(p)
  Demux4/3 -> Bus Creator/3  "shear_forcez"
  Rotation Angles to Direction Cosine Matrix1/1 -> Product2/1, Product1/1
  MATLAB Function2/1(F_b) -> Product1/2
  Demux2/3 -> Bus Creator1/6  "Bending_momenty"
  Demux6/1 -> Bus Creator2/4  "Torision_moment"
  Selector11/1 -> MATLAB Function2/2(M)
  Demux3/1 -> Bus Creator2/1  "Axial_Force"
  Product6/1 -> Demux4/1
  Mux/1 -> Gain/1
  Constant6/1 -> Mux/1
  Rotation Angles to Direction Cosine Matrix2/1 -> Product3/1, Product4/1
  Demux2/1 -> Bus Creator1/4  "Torision_moment"
  In1/1 -> Selector5/1, Selector1/1, Selector2/1
  Demux4/1 -> Bus Creator/1  "Axial_Force"
  Bus Creator/1 -> Bus Creator4/1
  Product7/1 -> Demux5/1
  Selector9/1 -> MATLAB Function1/1(F)
  Demux1/1 -> Bus Creator1/1  "Axial_Force"
  Product3/1 -> Demux3/1
  Bus Creator2/1 -> Bus Creator4/3
  Gain/1 -> Rotation Angles to Direction Cosine Matrix/1
  Constant2/1 -> Mux/3
  Demux5/1 -> Bus Creator/4  "Torision_moment"
  Constant1/1 -> MATLAB Function2/4(p)
  Selector5/1 -> Selector14/1, Selector13/1
  Demux5/3 -> Bus Creator/6  "Bending_momenty"
  Bus Creator1/1 -> Bus Creator4/2
  Selector12/1 -> MATLAB Function2/1(F)
  Demux4/2 -> Bus Creator/2  "shear_forcey"
  Selector1/1 -> Selector12/1, Selector11/1
  Demux5/2 -> Bus Creator/5  "Bending_momentx"
  Demux1/3 -> Bus Creator1/3  "shear_forcez"
  Selector6/1 -> MATLAB Function3/3(r)
  MATLAB Function1/1(F_b) -> Product6/2
  Demux6/3 -> Bus Creator2/6  "Bending_momenty"
  Demux1/2 -> Bus Creator1/2  "shear_forcey"
  MATLAB Function1/2(M_b) -> Product7/2
  MATLAB Function3/2(M_b) -> Product4/2
  Selector4/1 -> MATLAB Function2/3(r)
  Demux3/3 -> Bus Creator2/3  "shear_forcez"

== system aerodynamic_model_V1_2_Wrench/Load Estimator/Engine_station1/Subsystem4 ==
  In1 : Inport
  r_cg_up : Inport  Port=2
  Bus Creator : BusCreator  Inputs=6
  Bus Creator1 : BusCreator  Inputs=6
  Bus Creator2 : BusCreator  Inputs=6
  Bus Creator4 : BusCreator  Inputs=3
  Constant : Constant  Value=r_cg2node_b(:,79)
  Constant1 : Constant  Value=r_cg2node_b(:,78)
  Constant10 : Constant  Value=90
  Constant2 : Constant  Value=0
  Constant3 : Constant  Value=r_cg2node_b(:,47)
  Constant4 : Constant  Value=[0 0 0]/180*pi
  Constant5 : Constant  Value=[-7 0 0]/180*pi
  Constant6 : Constant  Value=-7
  Constant7 : Constant  Value=90
  Constant8 : Constant  Value=180
  Constant9 : Constant  Value=7
  Demux{1..6} (6 alike) : Demux  Outputs=3
  Display : Display
  Gain : Gain  Gain=pi/180
  Gain1 : Gain  Gain=pi/180
  MATLAB Function1 : MATLAB Function  TreatAsAtomicUnit=on
  MATLAB Function2 : MATLAB Function  TreatAsAtomicUnit=on
  MATLAB Function3 : MATLAB Function  TreatAsAtomicUnit=on
  Mux : Mux  Inputs=3
  Mux1 : Mux  Inputs=3
  Product{1..4,6..7} (6 alike) : Product  Multiplication=Matrix(*)
  Rotation Angles to Direction Cosine Matrix : Angle2Dcm  rotationOrder=XYZ
      settings: AttributesFormatString=Rotation Order: %<rotationOrder>
  Rotation Angles to Direction Cosine Matrix1 : Angle2Dcm  rotationOrder=XYZ
      settings: AttributesFormatString=Rotation Order: %<rotationOrder>
  Rotation Angles to Direction Cosine Matrix2 : Angle2Dcm  rotationOrder=XYZ
      settings: AttributesFormatString=Rotation Order: %<rotationOrder>
  Rotation Angles to Direction Cosine Matrix3 : Angle2Dcm  rotationOrder=ZXY
      settings: AttributesFormatString=Rotation Order: %<rotationOrder>
  Selector1 : Selector  NumberOfDimensions=2  InputPortWidth=3  IndexOptions=Select all,Index vector (dialog)  Indices=[1:6],[78 79]  OutputSizes=1,1
  Selector10 : Selector  NumberOfDimensions=2  InputPortWidth=3  IndexOptions=Index vector (dialog),Select all  Indices=[4:6],[surface_nodes.wing_R.node_id]  OutputSizes=1,1
  Selector11 : Selector  NumberOfDimensions=2  InputPortWidth=3  IndexOptions=Index vector (dialog),Select all  Indices=[4:6],[surface_nodes.wing_R.node_id]  OutputSizes=1,1
  Selector12 : Selector  NumberOfDimensions=2  InputPortWidth=3  IndexOptions=Index vector (dialog),Select all  Indices=[1:3],[surface_nodes.wing_R.node_id]  OutputSizes=1,1
  Selector13 : Selector  NumberOfDimensions=2  InputPortWidth=3  IndexOptions=Index vector (dialog),Select all  Indices=[4:6],[surface_nodes.wing_R.node_id]  OutputSizes=1,1
  Selector14 : Selector  NumberOfDimensions=2  InputPortWidth=3  IndexOptions=Index vector (dialog),Select all  Indices=[1:3],[surface_nodes.wing_R.node_id]  OutputSizes=1,1
  Selector2 : Selector  NumberOfDimensions=2  InputPortWidth=3  IndexOptions=Select all,Index vector (dialog)  Indices=[1:6],[79]  OutputSizes=1,1
  Selector3 : Selector  NumberOfDimensions=2  InputPortWidth=3  IndexOptions=Select all,Index vector (dialog)  Indices=[1:6],[79]  OutputSizes=1,1
  Selector5 : Selector  NumberOfDimensions=2  InputPortWidth=3  IndexOptions=Select all,Index vector (dialog)  Indices=[1:6],[77:79]  OutputSizes=1,1
  Selector6 : Selector  NumberOfDimensions=2  InputPortWidth=3  IndexOptions=Select all,Index vector (dialog)  Indices=[1:6],[77:79]  OutputSizes=1,1
  Selector7 : Selector  NumberOfDimensions=2  InputPortWidth=3  IndexOptions=Select all,Index vector (dialog)  Indices=[1:6],[78 79]  OutputSizes=1,1
  Selector9 : Selector  NumberOfDimensions=2  InputPortWidth=3  IndexOptions=Index vector (dialog),Select all  Indices=[1:3],[surface_nodes.wing_R.node_id]  OutputSizes=1,1
  Sum : Sum  Inputs=|++
  Out1 : Outport
  wires:
  Sum/1 -> Display/1
  Rotation Angles to Direction Cosine Matrix3/1 -> Sum/1
  Constant10/1 -> Mux1/2
  Mux1/1 -> Gain1/1
  Constant9/1 -> Mux1/1
  Gain1/1 -> Rotation Angles to Direction Cosine Matrix3/1
  Constant8/1 -> Mux1/3
  Demux3/3 -> Bus Creator2/3  "shear_forcez"
  Selector7/1 -> MATLAB Function2/3(r)
  MATLAB Function3/2(M_b) -> Product4/2
  MATLAB Function1/2(M_b) -> Product7/2
  Demux1/2 -> Bus Creator1/2  "shear_forcey"
  Demux6/3 -> Bus Creator2/6  "Bending_momenty"
  MATLAB Function1/1(F_b) -> Product6/2
  Selector6/1 -> MATLAB Function3/3(r)
  Demux1/3 -> Bus Creator1/3  "shear_forcez"
  Demux5/2 -> Bus Creator/5  "Bending_momentx"
  Selector1/1 -> Selector11/1, Selector12/1
  Demux4/2 -> Bus Creator/2  "shear_forcey"
  Selector12/1 -> MATLAB Function2/1(F)
  Bus Creator1/1 -> Bus Creator4/2
  Demux5/3 -> Bus Creator/6  "Bending_momenty"
  Selector5/1 -> Selector13/1, Selector14/1
  Constant1/1 -> MATLAB Function2/4(p)
  Demux5/1 -> Bus Creator/4  "Torision_moment"
  Constant2/1 -> Mux/3
  Gain/1 -> Rotation Angles to Direction Cosine Matrix/1
  Bus Creator2/1 -> Bus Creator4/3
  Product3/1 -> Demux3/1
  Demux1/1 -> Bus Creator1/1  "Axial_Force"
  Selector9/1 -> MATLAB Function1/1(F)
  Product7/1 -> Demux5/1
  Bus Creator/1 -> Bus Creator4/1
  Demux4/1 -> Bus Creator/1  "Axial_Force"
  In1/1 -> Selector5/1, Selector1/1, Selector2/1
  Demux2/1 -> Bus Creator1/4  "Torision_moment"
  Rotation Angles to Direction Cosine Matrix2/1 -> Product4/1, Product3/1
  Constant6/1 -> Mux/1
  Mux/1 -> Gain/1
  Product6/1 -> Demux4/1
  Demux3/1 -> Bus Creator2/1  "Axial_Force"
  Selector11/1 -> MATLAB Function2/2(M)
  Demux6/1 -> Bus Creator2/4  "Torision_moment"
  Demux2/3 -> Bus Creator1/6  "Bending_momenty"
  MATLAB Function2/1(F_b) -> Product1/2
  Rotation Angles to Direction Cosine Matrix1/1 -> Product1/1, Product2/1
  Demux4/3 -> Bus Creator/3  "shear_forcez"
  Constant3/1 -> MATLAB Function3/4(p)
  Product1/1 -> Demux1/1
  Product2/1 -> Demux2/1
  Constant5/1 -> Rotation Angles to Direction Cosine Matrix1/1
  MATLAB Function2/2(M_b) -> Product2/2
  Bus Creator4/1 -> Out1/1
  r_cg_up/1 -> Selector6/1, Selector7/1, Selector3/1
  Selector2/1 -> Selector10/1, Selector9/1
  MATLAB Function3/1(F_b) -> Product3/2
  Constant7/1 -> Mux/2
  Selector10/1 -> MATLAB Function1/2(M)
  Rotation Angles to Direction Cosine Matrix/1 -> Product7/1, Product6/1, Sum/2
  Selector13/1 -> MATLAB Function3/2(M)
  Constant4/1 -> Rotation Angles to Direction Cosine Matrix2/1
  Selector14/1 -> MATLAB Function3/1(F)
  Demux2/2 -> Bus Creator1/5  "Bending_momentx"
  Demux3/2 -> Bus Creator2/2  "shear_forcey"
  Selector3/1 -> MATLAB Function1/3(r)
  Constant/1 -> MATLAB Function1/4(p)
  Demux6/2 -> Bus Creator2/5  "Bending_momentx"
  Product4/1 -> Demux6/1

== system aerodynamic_model_V1_2_Wrench/Load Estimator/Engine_station1/Subsystem5 ==
  Wb_total : Inport
  r_cg_up : Inport  Port=2
  tilt_deg : Inport  Port=3
  Bus Creator : BusCreator  Inputs=6
  Bus Creator1 : BusCreator  Inputs=6
  Bus Creator2 : BusCreator  Inputs=6
  Bus Creator4 : BusCreator  Inputs=3
  Constant : Constant  Value=r_cg2node_b(:,73)
  Constant1 : Constant  Value=r_cg2node_b(:,72)
  Constant2 : Constant  Value=0
  Constant3 : Constant  Value=r_cg2node_b(:,29)
  Constant4 : Constant  Value=[0 0 0]/180*pi
  Constant5 : Constant  Value=[7 0 0]/180*pi
  Constant6 : Constant  Value=-7
  Demux{1..6} (6 alike) : Demux  Outputs=3
  Gain : Gain  Gain=pi/180
  MATLAB Function1 : MATLAB Function  TreatAsAtomicUnit=on
  MATLAB Function2 : MATLAB Function  TreatAsAtomicUnit=on
  MATLAB Function3 : MATLAB Function  TreatAsAtomicUnit=on
  Mux : Mux  Inputs=3
  Product{1..4,6..7} (6 alike) : Product  Multiplication=Matrix(*)
  Rotation Angles to Direction Cosine Matrix : Angle2Dcm  rotationOrder=XYZ
      settings: AttributesFormatString=Rotation Order: %<rotationOrder>
  Rotation Angles to Direction Cosine Matrix1 : Angle2Dcm  rotationOrder=XYZ
      settings: AttributesFormatString=Rotation Order: %<rotationOrder>
  Rotation Angles to Direction Cosine Matrix2 : Angle2Dcm  rotationOrder=XYZ
      settings: AttributesFormatString=Rotation Order: %<rotationOrder>
  Selector1 : Selector  NumberOfDimensions=2  InputPortWidth=3  IndexOptions=Select all,Index vector (dialog)  Indices=[1:6],[72 73]  OutputSizes=1,1
  Selector10 : Selector  NumberOfDimensions=2  InputPortWidth=3  IndexOptions=Index vector (dialog),Select all  Indices=[4:6],[surface_nodes.wing_R.node_id]  OutputSizes=1,1
  Selector11 : Selector  NumberOfDimensions=2  InputPortWidth=3  IndexOptions=Index vector (dialog),Select all  Indices=[4:6],[surface_nodes.wing_R.node_id]  OutputSizes=1,1
  Selector12 : Selector  NumberOfDimensions=2  InputPortWidth=3  IndexOptions=Index vector (dialog),Select all  Indices=[1:3],[surface_nodes.wing_R.node_id]  OutputSizes=1,1
  Selector13 : Selector  NumberOfDimensions=2  InputPortWidth=3  IndexOptions=Index vector (dialog),Select all  Indices=[4:6],[surface_nodes.wing_R.node_id]  OutputSizes=1,1
  Selector14 : Selector  NumberOfDimensions=2  InputPortWidth=3  IndexOptions=Index vector (dialog),Select all  Indices=[1:3],[surface_nodes.wing_R.node_id]  OutputSizes=1,1
  Selector2 : Selector  NumberOfDimensions=2  InputPortWidth=3  IndexOptions=Select all,Index vector (dialog)  Indices=[1:6],[73]  OutputSizes=1,1
  Selector3 : Selector  NumberOfDimensions=2  InputPortWidth=3  IndexOptions=Select all,Index vector (dialog)  Indices=[1:6],[73]  OutputSizes=1,1
  Selector4 : Selector  NumberOfDimensions=2  InputPortWidth=3  IndexOptions=Select all,Index vector (dialog)  Indices=[1:6],[72 73]  OutputSizes=1,1
  Selector5 : Selector  NumberOfDimensions=2  InputPortWidth=3  IndexOptions=Select all,Index vector (dialog)  Indices=[1:6],[71:73]  OutputSizes=1,1
  Selector6 : Selector  NumberOfDimensions=2  InputPortWidth=3  IndexOptions=Select all,Index vector (dialog)  Indices=[1:6],[71:73]  OutputSizes=1,1
  Selector9 : Selector  NumberOfDimensions=2  InputPortWidth=3  IndexOptions=Index vector (dialog),Select all  Indices=[1:3],[surface_nodes.wing_R.node_id]  OutputSizes=1,1
  Out1 : Outport
  wires:
  Product4/1 -> Demux6/1
  Demux6/2 -> Bus Creator2/5  "Bending_momentx"
  Constant/1 -> MATLAB Function1/4(p)
  Selector3/1 -> MATLAB Function1/3(r)
  Demux3/2 -> Bus Creator2/2  "shear_forcey"
  Demux2/2 -> Bus Creator1/5  "Bending_momentx"
  Selector14/1 -> MATLAB Function3/1(F)
  Constant4/1 -> Rotation Angles to Direction Cosine Matrix2/1
  Selector13/1 -> MATLAB Function3/2(M)
  Rotation Angles to Direction Cosine Matrix/1 -> Product6/1, Product7/1
  Selector10/1 -> MATLAB Function1/2(M)
  tilt_deg/1 -> Mux/2
  MATLAB Function3/1(F_b) -> Product3/2
  Selector2/1 -> Selector9/1, Selector10/1
  r_cg_up/1 -> Selector4/1, Selector6/1, Selector3/1
  Bus Creator4/1 -> Out1/1
  MATLAB Function2/2(M_b) -> Product2/2
  Constant5/1 -> Rotation Angles to Direction Cosine Matrix1/1
  Product2/1 -> Demux2/1
  Product1/1 -> Demux1/1
  Constant3/1 -> MATLAB Function3/4(p)
  Demux4/3 -> Bus Creator/3  "shear_forcez"
  Rotation Angles to Direction Cosine Matrix1/1 -> Product2/1, Product1/1
  MATLAB Function2/1(F_b) -> Product1/2
  Demux2/3 -> Bus Creator1/6  "Bending_momenty"
  Demux6/1 -> Bus Creator2/4  "Torision_moment"
  Selector11/1 -> MATLAB Function2/2(M)
  Demux3/1 -> Bus Creator2/1  "Axial_Force"
  Product6/1 -> Demux4/1
  Mux/1 -> Gain/1
  Constant6/1 -> Mux/1
  Rotation Angles to Direction Cosine Matrix2/1 -> Product3/1, Product4/1
  Demux2/1 -> Bus Creator1/4  "Torision_moment"
  Wb_total/1 -> Selector2/1, Selector5/1, Selector1/1
  Demux4/1 -> Bus Creator/1  "Axial_Force"
  Bus Creator/1 -> Bus Creator4/1
  Product7/1 -> Demux5/1
  Selector9/1 -> MATLAB Function1/1(F)
  Demux1/1 -> Bus Creator1/1  "Axial_Force"
  Product3/1 -> Demux3/1
  Bus Creator2/1 -> Bus Creator4/3
  Gain/1 -> Rotation Angles to Direction Cosine Matrix/1
  Constant2/1 -> Mux/3
  Demux5/1 -> Bus Creator/4  "Torision_moment"
  Constant1/1 -> MATLAB Function2/4(p)
  Selector5/1 -> Selector14/1, Selector13/1
  Demux5/3 -> Bus Creator/6  "Bending_momenty"
  Bus Creator1/1 -> Bus Creator4/2
  Selector12/1 -> MATLAB Function2/1(F)
  Demux4/2 -> Bus Creator/2  "shear_forcey"
  Selector1/1 -> Selector12/1, Selector11/1
  Demux5/2 -> Bus Creator/5  "Bending_momentx"
  Demux1/3 -> Bus Creator1/3  "shear_forcez"
  Selector6/1 -> MATLAB Function3/3(r)
  MATLAB Function1/1(F_b) -> Product6/2
  Demux6/3 -> Bus Creator2/6  "Bending_momenty"
  Demux1/2 -> Bus Creator1/2  "shear_forcey"
  MATLAB Function1/2(M_b) -> Product7/2
  MATLAB Function3/2(M_b) -> Product4/2
  Selector4/1 -> MATLAB Function2/3(r)
  Demux3/3 -> Bus Creator2/3  "shear_forcez"
